simulink model "Anuwa_Robotics"  (R2026a)
settings: Solver=FixedStepAuto  StopTime=inf  FixedStep=0.02
undefined symbols (not defined in the file): dspblkCoreblockFVToolHelper, gcbh, LF
libraries: dspstat3 x4, instrumentseriallib x2, dspxfrm3 x2, dspsigops x2, dspnetwork x1
settings Model: Creator=Deivis Paz  LastModifiedBy=Usuario Publico
settings OptimizationCC: PassReuseOutputArgsThreshold=0.0
settings HardwareCC: ProdLargestAtomicInteger=Long  ProdLargestAtomicFloat=Double  ProdHWDeviceType=ARM Compatible->ARM Cortex-M
settings RTWCC: GenCodeOnly=on  TargetLang=C++
settings GRTTargetCC: TargetLangStandard=C++03 (ISO)  CodeInterfacePackaging=C++ class  SubcomponentCodeInterfacePackaging=C++ class

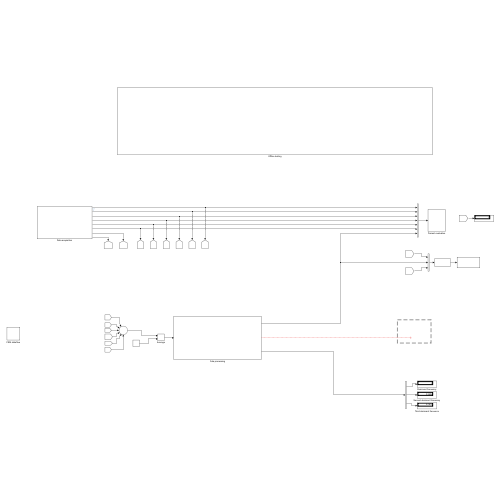
[thumbnail: Simulink's stored preview of the top-level diagram]
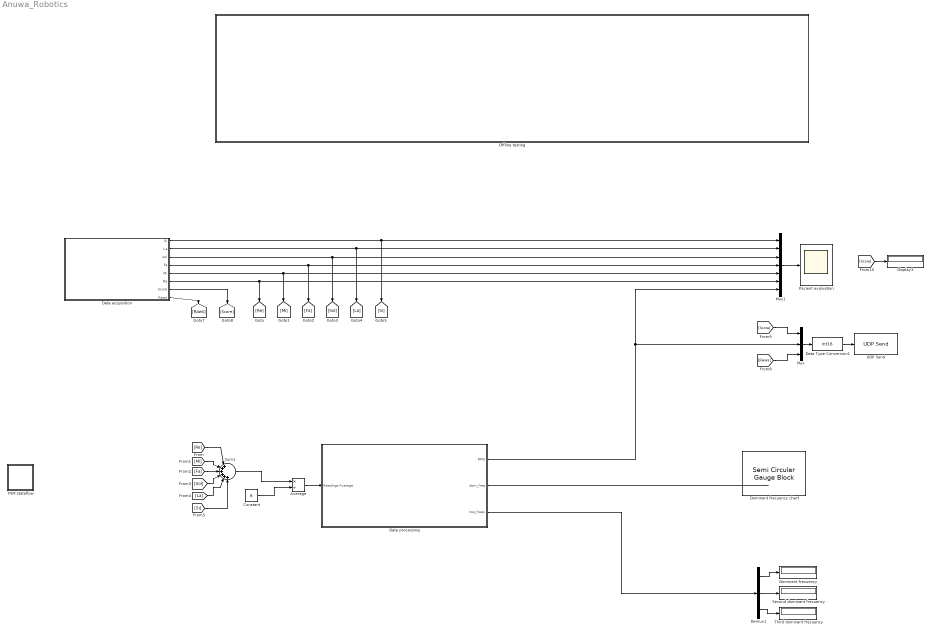
== system Anuwa_Robotics ==
  Average : Product  Inputs=*/
  Constant : Constant  Value=6
  Data Type Conversion1 : DataTypeConversion  OutDataTypeStr=int16  SaturateOnIntegerOverflow=off  RndMeth=Floor
  Data acquisition : Subsystem
  Data processing : Subsystem
  Demux1 : Demux  Outputs=3
  Display3 : Display
  Dominant frecuency : Display
  Dominant frecuency chart : SemiCircularGaugeBlock  ScaleMax=12  FontColor=[0.0, 0.0, 0.0]
  FSM stateflow : Subsystem  TreatAsAtomicUnit=on
  Mux : Mux  Inputs=3
  Mux1 : Mux  Inputs=7
  Offline testing : Subsystem
  Pacient evaluation : Scope
  Second dominant frecuency : Display
  Sum1 : Sum  Inputs=|++++++
  Third dominant frecuency : Display
  UDP Send : dspnetwork/UDP Send  remoteURL='127.0.0.1'  remotePort=5005  localURL='0.0.0.0'  localPortSource=Automatically determine  localPort=-1  sendBufferSize=8192  sampletime=-1  blockPlatform=[]  separateLengthPort=0
      settings: LibrarySourceBlock=dspsnks4/UDP Send
  wires:
  Demux1/1 -> Dominant frecuency/1
  Demux1/2 -> Second dominant frecuency/1
  Demux1/3 -> Third dominant frecuency/1
  Mux/1 -> Data Type Conversion1/1
  Data Type Conversion1/1 -> UDP Send/1
  Data acquisition/2(La) -> Mux1/2, [La]
  Data acquisition/5(Mi) -> Mux1/5, [Mi]
  Data acquisition/6(Re) -> Mux1/6, [Re]
  Data acquisition/3(sol) -> Mux1/3, [Sol]
  Data acquisition/4(fa) -> Mux1/4, [Fa]
  Data acquisition/1(Si) -> Mux1/1, [Si]
  Data acquisition/7(Score) -> [Score]
  Sum1/1 -> Average/1
  Constant/1 -> Average/2
  Mux1/1 -> Pacient evaluation/1
  [Re] -> Sum1/1
  [Mi] -> Sum1/2
  [Fa] -> Sum1/3
  [Sol] -> Sum1/4
  [La] -> Sum1/5
  [Si] -> Sum1/6
  Data acquisition/8(Raws) -> [Raws]
  [Raws] -> Mux/3
  [Score] -> Mux/1
  [Score] -> Display3/1
  Data processing/1(RMS) -> Mux/2, Mux1/7
  Average/1 -> Data processing/1(Readings Average)
  Data processing/3(top_freqs) -> Demux1/1
  Data processing/2(dom_freq) -> ?

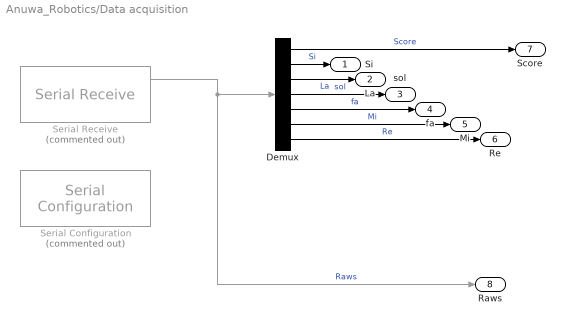
== system Anuwa_Robotics/Data acquisition ==
  Demux : Demux  Outputs=7
  Serial Configuration : instrumentseriallib/Serial Configuration  Priority=-200000  Commented=on  PortSel=<Select a port...>  Port=<Select a port...>  ComPort=<Select a port...>  BaudRate=115200  DataBits=8  Parity=none  StopBits=1  ByteOrder=little-endian  FlowControl=none  Timeout=10  SimulateUsing=Interpreted execution  BlockInModel=on  aMode=1
  Serial Receive : instrumentseriallib/Serial Receive  Priority=1  Commented=on  PortSel=<Select a port...>  Port=<Select a port...>  ComPort=<Select a port...>  DataType=int16  SaveDataType=uint8  ToggleHeader=on  Header=[0xAA, 0xBB]  ToggleDataSize=on  DataSize=[8]  ToggleTerminator=off  Terminator=LF ('\n')  CustomTerminator=[]  InputFormat=Column major  EnableBlockingMode=off  ActionDataUnavailable=Output last received value  ActionWhenDataUnavailable=Output last received value  CustomValue=0  SampleTime=0.02  SimulateUsing=Interpreted execution  BlockInModel=on  aMode=1  LibraryInUse=instrumentlib
  Si : Outport
  La : Outport  Port=2
  sol : Outport  Port=3
  fa : Outport  Port=4
  Mi : Outport  Port=5
  Re : Outport  Port=6
  Score : Outport  Port=7
  Raws : Outport  Port=8
  wires:
  Demux/3 -> La/1  "La"
  Demux/1 -> Score/1  "Score"
  Serial Receive/1 -> Raws/1, Demux/1  "Raws"
  Demux/6 -> Mi/1  "Mi"
  Demux/7 -> Re/1  "Re"
  Demux/5 -> fa/1  "fa"
  Demux/4 -> sol/1  "sol"
  Demux/2 -> Si/1  "Si"

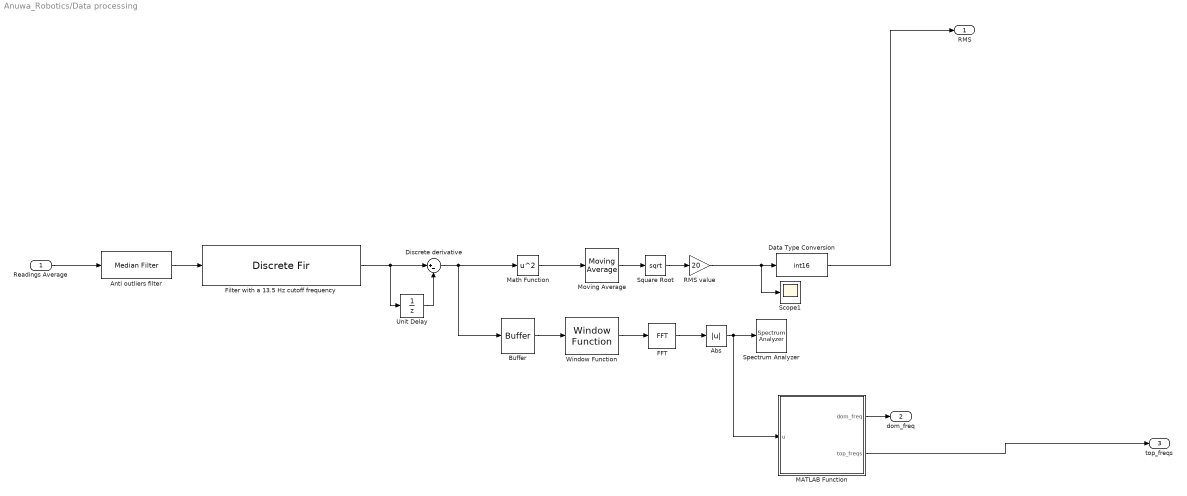
== system Anuwa_Robotics/Data processing ==
  Readings Average : Inport
  Abs : Abs  SaturateOnIntegerOverflow=off
  Anti outliers filter : dspstat3/Median Filter  WindowLength=3  SimulateUsing=Interpreted execution
      settings: LibrarySourceBlock=|
      | dspfdesign/Median
      | Filter
  Buffer : Buffer  N=128  V=96  OutputFrames=off
  Data Type Conversion : DataTypeConversion  OutDataTypeStr=int16  SaturateOnIntegerOverflow=off  RndMeth=Floor
  Discrete derivative : Sum  Inputs=|+-
  FFT : dspxfrm3/FFT  FFTImplementation=Auto  CompMethod=Table lookup  TableOpt=NEW  TableOptActive=Speed  BitRevOrder=off  Normalize=off  InheritFFTLength=on  FFTLength=64  WrapInput=on  roundingMode=Ceiling  overflowMode=off  firstCoeffDataTypeStr=Inherit: Same word length as input  firstCoeffLastDataTypeStr=Inherit: Same word length as input  outputMin=[]  outputMax=[]
  Filter with a 13.5 Hz cutoff frequency : DiscreteFir  LoadFcn=dspblkCoreblockFVToolHelper(gcbh,'load');  Coefficients=[0.000122839826262800, -0.001062043534259923, 0.000155311501942401, 0.001474122429057481, -0.000707240877932949, -0.002145707147559719, 0.001831903785886181, 0.002871521633811274, -0.003800017837134007, -0.003275308198022955, 0.006789018842957049, 0.002821173563717651, -0.010829494430763456, -0.000830808237550620, 0.015774668999938995, -0.003527444496181349, -0.021300559192349085, 0.011358963820317883, 0.026938779886598509, -0.024511060541039839, -0.032137742199404698, 0.047343180110038151, 0.036342380526401256, -0.095770876785395975, -0.039078706552677915, 0.314962724817361706, 0.540380840571962340, 0.314962724817361706, -0.039078706552677915, -0.095770876785395975, 0.036342380526401263, 0.047343180110038165, -0.032137742199404698, -0.024511060541039843, 0.026938779886598513, 0.011358963820317884, -0.021300559192349088, -0.003527444496181350, 0.015774668999939002, -0.000830808237550620, -0.010829494430763456, 0.002821173563717653, 0.006789018842957049, -0.003275308198022958, -0.003800017837134014, 0.002871521633811275, 0.001831903785886183, -0.002145707147559719, -0.000707240877932949, 0.001474122429057482, 0.000155311501942401, -0.001062043534259923, 0.000122839826262800]
      settings: CopyFcn=dspblkCoreblockFVToolHelper(gcbh,'copy');  DeleteFcn=dspblkCoreblockFVToolHelper(gcbh,'close');  ModelCloseFcn=dspblkCoreblockFVToolHelper(gcbh,'close');  PreSaveFcn=dspblkCoreblockFVToolHelper(gcbh,'presave');  PostSaveFcn=dspblkCoreblockFVToolHelper(gcbh,'postsave');  CloseFcn=dspblkCoreblockFVToolHelper(gcbh,'close');
  MATLAB Function : MATLAB Function  TreatAsAtomicUnit=on
  Math Function : Math  Operator=square  OutDataTypeStr=Inherit: Inherit via internal rule
  Moving Average : dspstat3/Moving Average  Method=Sliding window  ForgettingFactorPort=off  SpecifyWindowLength=on  WindowLengthSource=Property  MaxWindowLength=20  WindowLength=3  OverlapLength=2  AllowArbitraryInputLength=off  ForgettingFactor=0.9  SimulateUsing=Interpreted execution
  RMS value : Gain  Gain=20
  Scope1 : Scope
      settings: ActiveDisplayYMinimum=-1  ActiveDisplayYMaximum=1
  Spectrum Analyzer : SpectrumAnalyzer  WindowPosition=[598.000000,284.000000,800.000000,500.000000,]  ScopeFrameLocation=window  SampleRateSource=Property  SampleRate=50  PlotAsTwoSidedSpectrum=off  WindowInvariantSamplesPerUpdate=on  Span=25  CenterFrequency=12.5  StartFrequency=0  StopFrequency=25  YLimits=[-3603.4449 -2802.6794]
  Square Root : Sqrt
  Unit Delay : UnitDelay  SampleTime=0.02
  Window Function : dspsigops/Window Function  winmode=Apply window to input  wintype=Hamming  sampmode=Continuous  samptime=1  N=64  Rs=50  beta=10  winsamp=Symmetric  UserWindow=hamming  OptParams=off  UserParams={'symmetric'}  dataType=double  isSigned=on  wordLen=16  udDataType=sfix(16)  fracBitsMode=Best precision  numFracBits=15  roundingMode=Floor  overflowMode=off  numSidelobes=4  sidelobeLevel=-30
  RMS : Outport
  dom_freq : Outport  Port=2
  top_freqs : Outport  Port=3
  wires:
  Unit Delay/1 -> Discrete derivative/2
  Filter with a 13.5 Hz cutoff frequency/1 -> Discrete derivative/1, Unit Delay/1
  Square Root/1 -> RMS value/1
  Buffer/1 -> Window Function/1
  Discrete derivative/1 -> Buffer/1, Math Function/1
  Math Function/1 -> Moving Average/1
  RMS value/1 -> Scope1/1, Data Type Conversion/1
  FFT/1 -> Abs/1
  Moving Average/1 -> Square Root/1
  Window Function/1 -> FFT/1
  MATLAB Function/2(top_freqs) -> top_freqs/1
  Abs/1 -> MATLAB Function/1(u), Spectrum Analyzer/1
  Readings Average/1 -> Anti outliers filter/1
  Data Type Conversion/1 -> RMS/1
  MATLAB Function/1(dom_freq) -> dom_freq/1
  Anti outliers filter/1 -> Filter with a 13.5 Hz cutoff frequency/1

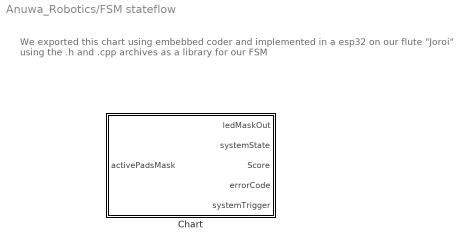
== system Anuwa_Robotics/FSM stateflow ==
  note: We exported this chart using embebbed coder and implemented in a esp32 on our flute "Joroi" using the .h and .cpp archives as a library for our FSM
  Chart : Stateflow chart  TreatAsAtomicUnit=on

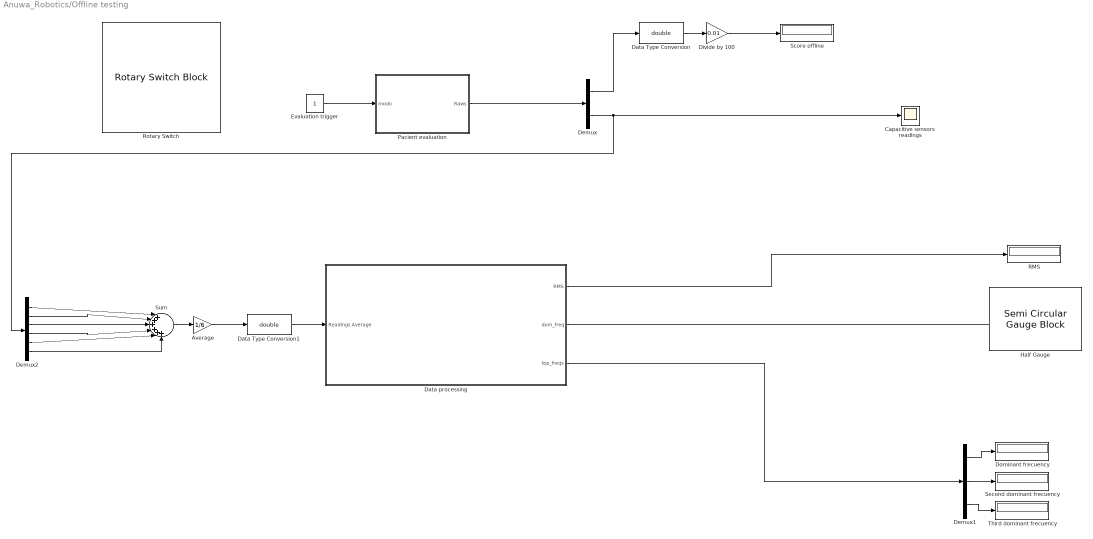
== system Anuwa_Robotics/Offline testing ==
  Average : Gain  Gain=1/6
  Capacitive sensors readings : Scope
      settings: ActiveDisplayYMinimum=-21.284308306767471  ActiveDisplayYMaximum=108.7467943389273  DataLoggingVariableName=ScopeData2
  Data Type Conversion : DataTypeConversion  OutDataTypeStr=double  SaturateOnIntegerOverflow=off  RndMeth=Floor
  Data Type Conversion1 : DataTypeConversion  OutDataTypeStr=double  SaturateOnIntegerOverflow=off  RndMeth=Floor
  Data processing : Subsystem
  Demux : Demux  Outputs=[1 6]
  Demux1 : Demux  Outputs=3
  Demux2 : Demux  Outputs=6
  Divide by 100 : Gain  Gain=0.01
  Dominant frecuency : Display
  Evaluation trigger : Constant  SampleTime=0.02
  Half Gauge : SemiCircularGaugeBlock  ScaleMax=12  FontColor=[0.0, 0.0, 0.0]
  Pacient evaluation : MATLAB Function  TreatAsAtomicUnit=on
  RMS : Display
  Rotary Switch : RotarySwitchBlock
  Score offline : Display
  Second dominant frecuency : Display
  Sum : Sum  Inputs=|++++++
  Third dominant frecuency : Display
  wires:
  Demux/2 -> Demux2/1, Capacitive sensors readings/1
  Demux/1 -> Data Type Conversion/1
  Divide by 100/1 -> Score offline/1
  Data Type Conversion/1 -> Divide by 100/1
  Evaluation trigger/1 -> Pacient evaluation/1(modo)
  Data processing/2(dom_freq) -> ?
  Demux1/3 -> Third dominant frecuency/1
  Demux1/1 -> Dominant frecuency/1
  Demux1/2 -> Second dominant frecuency/1
  Data processing/3(top_freqs) -> Demux1/1
  Data processing/1(RMS) -> RMS/1
  Demux2/1 -> Sum/1
  Demux2/2 -> Sum/2
  Demux2/3 -> Sum/3
  Demux2/4 -> Sum/4
  Demux2/5 -> Sum/5
  Demux2/6 -> Sum/6
  Sum/1 -> Average/1
  Data Type Conversion1/1 -> Data processing/1(Readings Average)
  Average/1 -> Data Type Conversion1/1
  Pacient evaluation/1(Raws) -> Demux/1

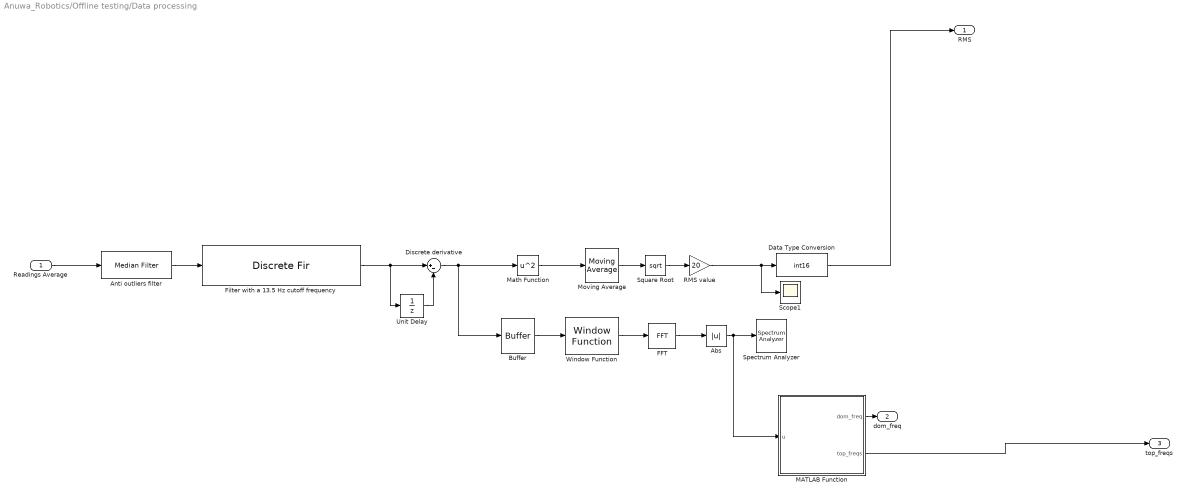
== system Anuwa_Robotics/Offline testing/Data processing ==
  Readings Average : Inport
  Abs : Abs  SaturateOnIntegerOverflow=off
  Anti outliers filter : dspstat3/Median Filter  WindowLength=3  SimulateUsing=Interpreted execution
      settings: LibrarySourceBlock=|
      | dspfdesign/Median
      | Filter
  Buffer : Buffer  N=128  V=96  OutputFrames=off
  Data Type Conversion : DataTypeConversion  OutDataTypeStr=int16  SaturateOnIntegerOverflow=off  RndMeth=Floor
  Discrete derivative : Sum  Inputs=|+-
  FFT : dspxfrm3/FFT  FFTImplementation=Auto  CompMethod=Table lookup  TableOpt=NEW  TableOptActive=Speed  BitRevOrder=off  Normalize=off  InheritFFTLength=on  FFTLength=64  WrapInput=on  roundingMode=Ceiling  overflowMode=off  firstCoeffDataTypeStr=Inherit: Same word length as input  firstCoeffLastDataTypeStr=Inherit: Same word length as input  outputMin=[]  outputMax=[]
  Filter with a 13.5 Hz cutoff frequency : DiscreteFir  LoadFcn=dspblkCoreblockFVToolHelper(gcbh,'load');  Coefficients=[0.000122839826262800, -0.001062043534259923, 0.000155311501942401, 0.001474122429057481, -0.000707240877932949, -0.002145707147559719, 0.001831903785886181, 0.002871521633811274, -0.003800017837134007, -0.003275308198022955, 0.006789018842957049, 0.002821173563717651, -0.010829494430763456, -0.000830808237550620, 0.015774668999938995, -0.003527444496181349, -0.021300559192349085, 0.011358963820317883, 0.026938779886598509, -0.024511060541039839, -0.032137742199404698, 0.047343180110038151, 0.036342380526401256, -0.095770876785395975, -0.039078706552677915, 0.314962724817361706, 0.540380840571962340, 0.314962724817361706, -0.039078706552677915, -0.095770876785395975, 0.036342380526401263, 0.047343180110038165, -0.032137742199404698, -0.024511060541039843, 0.026938779886598513, 0.011358963820317884, -0.021300559192349088, -0.003527444496181350, 0.015774668999939002, -0.000830808237550620, -0.010829494430763456, 0.002821173563717653, 0.006789018842957049, -0.003275308198022958, -0.003800017837134014, 0.002871521633811275, 0.001831903785886183, -0.002145707147559719, -0.000707240877932949, 0.001474122429057482, 0.000155311501942401, -0.001062043534259923, 0.000122839826262800]
      settings: CopyFcn=dspblkCoreblockFVToolHelper(gcbh,'copy');  DeleteFcn=dspblkCoreblockFVToolHelper(gcbh,'close');  ModelCloseFcn=dspblkCoreblockFVToolHelper(gcbh,'close');  PreSaveFcn=dspblkCoreblockFVToolHelper(gcbh,'presave');  PostSaveFcn=dspblkCoreblockFVToolHelper(gcbh,'postsave');  CloseFcn=dspblkCoreblockFVToolHelper(gcbh,'close');
  MATLAB Function : MATLAB Function  TreatAsAtomicUnit=on
  Math Function : Math  Operator=square  OutDataTypeStr=Inherit: Inherit via internal rule
  Moving Average : dspstat3/Moving Average  Method=Sliding window  ForgettingFactorPort=off  SpecifyWindowLength=on  WindowLengthSource=Property  MaxWindowLength=20  WindowLength=3  OverlapLength=2  AllowArbitraryInputLength=off  ForgettingFactor=0.9  SimulateUsing=Interpreted execution
  RMS value : Gain  Gain=20
  Scope1 : Scope
      settings: ActiveDisplayYMinimum=-1  ActiveDisplayYMaximum=1
  Spectrum Analyzer : SpectrumAnalyzer  WindowPosition=[380.000000,40.000000,800.000000,500.000000,]  ScopeFrameLocation=window  SampleRateSource=Property  SampleRate=50  PlotAsTwoSidedSpectrum=off  WindowInvariantSamplesPerUpdate=on  Span=25  CenterFrequency=12.5  StartFrequency=0  StopFrequency=25  YLimits=[-23.8659 56.0559]
  Square Root : Sqrt
  Unit Delay : UnitDelay  SampleTime=0.02
  Window Function : dspsigops/Window Function  winmode=Apply window to input  wintype=Hamming  sampmode=Continuous  samptime=1  N=64  Rs=50  beta=10  winsamp=Symmetric  UserWindow=hamming  OptParams=off  UserParams={'symmetric'}  dataType=double  isSigned=on  wordLen=16  udDataType=sfix(16)  fracBitsMode=Best precision  numFracBits=15  roundingMode=Floor  overflowMode=off  numSidelobes=4  sidelobeLevel=-30
  RMS : Outport
  dom_freq : Outport  Port=2
  top_freqs : Outport  Port=3
  wires:
  Unit Delay/1 -> Discrete derivative/2
  Filter with a 13.5 Hz cutoff frequency/1 -> Discrete derivative/1, Unit Delay/1
  Square Root/1 -> RMS value/1
  Buffer/1 -> Window Function/1
  Discrete derivative/1 -> Buffer/1, Math Function/1
  Math Function/1 -> Moving Average/1
  RMS value/1 -> Scope1/1, Data Type Conversion/1
  FFT/1 -> Abs/1
  Moving Average/1 -> Square Root/1
  Window Function/1 -> FFT/1
  MATLAB Function/2(top_freqs) -> top_freqs/1
  Abs/1 -> MATLAB Function/1(u), Spectrum Analyzer/1
  Readings Average/1 -> Anti outliers filter/1
  Data Type Conversion/1 -> RMS/1
  MATLAB Function/1(dom_freq) -> dom_freq/1
  Anti outliers filter/1 -> Filter with a 13.5 Hz cutoff frequency/1

== matlab function Anuwa_Robotics/Offline testing/Data processing/MATLAB Function ==
  data: u input; dom_freq output; top_freqs output
function [dom_freq, top_freqs] = procesar_fft(u)
    Fs = 50;
    N = length(u);
    half_N = floor(N/2);
    mag = u(1:half_N);
    mag(1) = 0;
    freqs = (0:half_N-1)' * (Fs/N);
    
    valid_idx = freqs <= 12;
    valid_freqs = freqs(valid_idx);
    valid_mag = mag(valid_idx);
    
    [~, sorted_idx] = sort(valid_mag, 'descend');
    
    top_freqs = zeros(3,1);
    if length(sorted_idx) >= 3
        top_freqs(1) = valid_freqs(sorted_idx(1));
        top_freqs(2) = valid_freqs(sorted_idx(2));
        top_freqs(3) = valid_freqs(sorted_idx(3));
    end
    
    if ~isempty(sorted_idx)
        dom_freq = valid_freqs(sorted_idx(1));
    else
        dom_freq = 0;
    end
end

== matlab function Anuwa_Robotics/Data processing/MATLAB Function ==
  data: u input; dom_freq output; top_freqs output
function [dom_freq, top_freqs] = procesar_fft(u)
    Fs = 50;
    N = length(u);
    half_N = floor(N/2);
    mag = u(1:half_N);
    mag(1) = 0;
    freqs = (0:half_N-1)' * (Fs/N);
    
    valid_idx = freqs <= 12;
    valid_freqs = freqs(valid_idx);
    valid_mag = mag(valid_idx);
    
    [~, sorted_idx] = sort(valid_mag, 'descend');
    
    top_freqs = zeros(3,1);
    if length(sorted_idx) >= 3
        top_freqs(1) = valid_freqs(sorted_idx(1));
        top_freqs(2) = valid_freqs(sorted_idx(2));
        top_freqs(3) = valid_freqs(sorted_idx(3));
    end
    
    if ~isempty(sorted_idx)
        dom_freq = valid_freqs(sorted_idx(1));
    else
        dom_freq = 0;
    end
end

== matlab function Anuwa_Robotics/Offline testing/Pacient evaluation ==
  data: Raws output; modo input
function Raws = simular_pacientes(modo)
    coder.extrinsic('pause');
    persistent tick modo_anterior
    if isempty(tick)
        tick = int32(0);
        modo_anterior = int32(0);
    end

    if int32(modo) ~= modo_anterior
        tick = int32(0);
        modo_anterior = int32(modo);
    end

    Raws = zeros(7, 1, 'int16');
    ticks_por_paso = int32(10);

    if modo == 1
        masks = uint8([0,0,0,0,0,0,0,0,0,0,1,3,3,1,1,1,1,0,1,1,1,1,1,1,1,3,3,3,3,3,3,3,3,3,3,3,3,15,15,15,15,15,31,31,31,31,31,31,31,31,31,7,7,7,0,0,0,0,0,0,0,0,0,0,3,3,3,3,3,3,3,3,3,1,1,1,3,3,1,1,1,1,1,1,1,1,1,3,3,3,3,3,3,3,3,1,1,1,1,3,3,3,3,3,3,3,3,3,3,3,3,3,3,3,3]);
        scores = int16([5000,5000,5000,5000,5000,5000,5000,5000,5000,5000,4800,4550,4250,3900,3950,4000,4050,3900,4020,4140,4260,4380,4180,3930,4050,4100,4150,4200,4250,4370,4490,4610,4730,4850,4970,5090,5210,5260,5380,5500,5620,5740,5860,5980,6100,6220,6340,6460,6580,6700,6820,6870,6920,7040,6890,6890,6890,6890,6890,6890,6890,6890,6890,6890,6690,6440,6140,6260,6380,6500,6620,6670,6720,6840,6960,7080,7130,6930,7050,7170,7290,7410,7530,7650,7770,7890,8010,8060,8180,8300,8420,8540,8660,8780,8900,8950,9070,9190,9310,9360,9480,9600,9720,9840,9960,10000,10000,10000,10000,10000,10000,10000,10000,10000,10000]);

        step_idx = idivide(tick, ticks_por_paso) + 1;
        if step_idx > 115
            pause(1.0);
            Raws(1) = scores(115);
            for i = 1:6
                Raws(i + 1) = int16(70 + i * 2);
            end
            return;
        end

        pause(0.02);
        t = double(tick) * 0.02;
        osc = int16(round(2.0 * sin(2 * pi * 1.5 * t) + 1.0 * cos(2 * pi * 2.2 * t)));

        m = masks(step_idx);
        Raws(1) = scores(step_idx);

        for i = 1:6
            if bitand(m, bitshift(uint8(1), i - 1)) > 0
                Raws(i + 1) = int16(15 + i * 2) + osc;
            else
                Raws(i + 1) = int16(70 + i * 2) + osc;
            end
        end
        tick = tick + 1;

    elseif modo == 2
        masks = uint8([0,0,1,1,1,1,1,1,1,1,0,0,1,2,1,1,1,1,1,4,0,0,0,0,1,1,1,0,0,1,3,1,0,2,0,3,2,1,2,4,5,3,0,3,1,3,3,7,7,7,7,7,9,15,11,1,1,25,57,57,0,0,0,0,1,1,1,3,3,1,0,1,0,16,16,0,0,1,0,8,8,40,56,56,56,24,0,1,1,1,0,6,8,16,27,1,8,11,8,9,8,0,0,2,0,1,1,1,1,1,2,0,2,2,0]);
        scores = int16([5000,5000,4800,4550,4250,3900,3500,3050,2550,2000,2000,2000,1800,1550,1600,1650,1700,1820,1940,1990,1840,1640,1640,1640,1760,1880,2000,1850,1650,1700,1820,1870,1720,1770,1620,1740,1790,1840,1890,1940,1990,2040,1890,1940,1990,2040,2090,2140,2190,2240,2290,2340,2390,2440,2490,2290,2040,1740,1390,990,990,990,990,990,790,540,240,360,480,530,380,500,350,400,450,300,100,0,0,50,100,150,200,250,300,350,200,320,370,420,270,320,370,420,470,520,570,620,670,720,770,620,420,470,320,370,420,470,520,570,620,470,520,570,420]);

        step_idx = idivide(tick, ticks_por_paso) + 1;
        if step_idx > 115
            pause(1.0);
            Raws(1) = scores(115);
            for i = 1:6
                Raws(i + 1) = int16(65 + i * 2);
            end
            return;
        end

        pause(0.02);
        t = double(tick) * 0.02;
        tremor = int16(round(14.0 * sin(2 * pi * 6.5 * t) + 8.0 * sin(2 * pi * 9.2 * t) + 5.0 * cos(2 * pi * 4.8 * t)));

        m = masks(step_idx);
        Raws(1) = scores(step_idx);

        for i = 1:6
            if bitand(m, bitshift(uint8(1), i - 1)) > 0
                Raws(i + 1) = int16(20 + i * 2) + tremor;
            else
                Raws(i + 1) = int16(65 + i * 2) + tremor;
            end
        end
        tick = tick + 1;

    else
        pause(1.0);
        Raws(1) = int16(5000);
        for i = 1:6
            Raws(i + 1) = int16(70 + i * 2);
        end
    end
end

== stateflow chart Anuwa_Robotics/FSM stateflow/Chart ==
  state STANDBY_TELEMETRY
    en:
    systemState = 0;
    systemTrigger = false;
    Score = 50.0;
    errorCode = 0;
    state Idle
      du: ledMaskOut = activePadsMask;
    state Hold
      du: ledMaskOut = activePadsMask;
    (default) -> Idle
    Hold -> Idle [order 1] : [activePadsMask ~= 56]
    Idle -> Hold : [activePadsMask == 56]
  state INIT_SEQUENCE
    en:
    systemState = 1;
    animStep = 0;
    state LED_SWEEP_ANIMATION
      en:
      ledMaskOut = uint8(bitshift(1, animStep));
      animStep = mod(animStep + 1, 6);
    (default) -> LED_SWEEP_ANIMATION
    LED_SWEEP_ANIMATION -> LED_SWEEP_ANIMATION : [after(60, msec)]
  state THERAPY_EXECUTION
    en:
    systemState = 2;
    executionStep = 0;
    touchCount = 0;
    omissionStreak = 0;
    ghostStreak = 0;
    ledMaskOut = 0;
    state WAIT_START
    state TOUCH_DETECTED
      en:
      touchCount = touchCount + 1;
    state TRIGGER_ORCHESTRA
      en:
      systemTrigger = true;
      executionStep = 4;
      ex:
      systemTrigger = false;
    state WAIT_RELEASE
    state GAME_LOOP
      en:
      [Score, errorCode, omissionStreak, ghostStreak] = calculatePrecision(activePadsMask, executionStep, Score, omissionStreak, ghostStreak);
      ledMaskOut = getPatternLeds(executionStep);
      executionStep = executionStep + 1;
    (default) -> WAIT_START
    WAIT_RELEASE -> WAIT_START : [activePadsMask == 0]
    WAIT_START -> TOUCH_DETECTED : [activePadsMask > 0]
    TOUCH_DETECTED -> TRIGGER_ORCHESTRA [order 2] : [touchCount == 4]
    TOUCH_DETECTED -> WAIT_RELEASE [order 1] : [touchCount < 4]
    TRIGGER_ORCHESTRA -> GAME_LOOP : [after(206, msec)]
    GAME_LOOP -> GAME_LOOP : [after(206, msec)]
  (default) -> STANDBY_TELEMETRY
  Hold -> INIT_SEQUENCE [order 2] : [after(300, msec)]
  INIT_SEQUENCE -> THERAPY_EXECUTION : [after(3, sec)]
  THERAPY_EXECUTION -> STANDBY_TELEMETRY : [executionStep >= 130]
  data: step function_input; ledMask function_output; receivedMask function_input; step function_input; energyIn function_input; omissionStreakIn function_input; ghostStreakIn function_input; energyOut function_output; errCode function_output; omissionStreakOut function_output; ghostStreakOut function_output; activePadsMask input uint8; ledMaskOut output uint8; systemState output uint8; Score output single; errorCode output int32; systemTrigger output boolean; animStep local int32; executionStep local int32; touchCount local int32; omissionStreak local int32; ghostStreak local int32
  function ledMask = getPatternLeds(step):
    | function ledMask = getPatternLeds(step)
    |     persistent pattern;
    |     if isempty(pattern)
    |         pattern = zeros(1, 130, 'uint8');
    |         
    |         valores = uint8([0, 0, 0, 0, 1, 1, 1, 1, 1, 1, 1, 1, 1, 1, 1, 1, 1, 7, 7, 3, 3, 3, 3, 3, 3, 1, 1, 3, 3, 3, 3, 3, 3, 3, 3, 3, 7, 7, 7, 7, 7, 7, 7, 7, 7, 7, 31, 31, 31, 31, 31, 63, 63, 63, 63, 63, 63, 63, 63, 63, 63, 63, 59, 1, 1, 1, 1, 1, 1, 1, 1, 1, 1, 1, 1, 1, 7, 7, 7, 3, 3, 3, 3, 3, 1, 1, 3, 3, 3, 3, 3, 3, 3, 3, 3, 7, 7, 7, 7, 7, 7, 7, 7, 3, 3, 3, 3, 3, 3, 7, 7, 7, 7, 7, 7]);
    |         
    |         for i = 1:length(valores)
    |             pattern(i) = valores(i);
    |         end
    |     end
    |     
    |     if step < 130
    |         ledMask = pattern(step + 1);
    |     else
    |         ledMask = uint8(0);
    |     end
    | end
  function [energyOut, errCode, omissionStreakOut, ghostStreakOut] = calculatePrecision(receivedMask, step, energyIn, omissionStreakIn, ghostStreakIn):
    | function [energyOut, errCode, omissionStreakOut, ghostStreakOut] = calculatePrecision(receivedMask, step, energyIn, omissionStreakIn, ghostStreakIn)
    |     energyOut = single(energyIn);
    |     errCode = int32(0);
    |     omissionStreakOut = int32(omissionStreakIn);
    |     ghostStreakOut = int32(ghostStreakIn);
    | 
    |     expectedMask = getPatternLeds(step);
    |     
    |     if expectedMask > 0
    |         if receivedMask == 0
    |             errCode = int32(1); 
    |             omissionStreakOut = omissionStreakOut + int32(1);
    |             ghostStreakOut = int32(0);
    |             energyOut = energyOut - single(1.0 + (single(omissionStreakOut) * 0.5));
    |         else
    |             omissionStreakOut = int32(0);
    |             ghostStreakOut = int32(0);
    |             if receivedMask == expectedMask
    |                 energyOut = energyOut + single(1.2); 
    |                 errCode = int32(0);
    |             else
    |                 energyOut = energyOut + single(0.5); 
    |                 errCode = int32(2);
    |             end
    |         end
    |     else
    |         if receivedMask > 0
    |             errCode = int32(3); 
    |             ghostStreakOut = ghostStreakOut + int32(1);
    |             omissionStreakOut = int32(0);
    |             energyOut = energyOut - single(1.5 + (single(ghostStreakOut) * 0.5));
    |         else
    |             errCode = int32(0);
    |             omissionStreakOut = int32(0);
    |             ghostStreakOut = int32(0);
    |         end
    |     end
    | 
    |     if energyOut > single(100.0)
    |         energyOut = single(100.0);
    |     elseif energyOut < single(0.0)
    |         energyOut = single(0.0);
    |     end
    | end
